simulink model "DATA_PERTURB_AND_OBSERVE_SOLAR_TRACKER"  (R2023b)
settings: Solver=ode23  StartTime=0.0  StopTime=12  RelTol=1e-7
undefined symbols (not defined in the file): Acid, Lead
libraries: spsMeanLib x5, spsSeriesRLCBranchLib x5, spsVoltageMeasurementLib x4, spsCurrentMeasurementLib x2, spsBatteryLib x1, spsDiodeLib x1, spsMosfetLib x1, simulink x1, spsPVArrayLib x1, spsPWMGeneratorDCDCLib x1, sps_lib x1
settings Model: Creator=User  LastModifiedBy=D E L L
settings DebuggingCC: AlgebraicLoopMsg=none

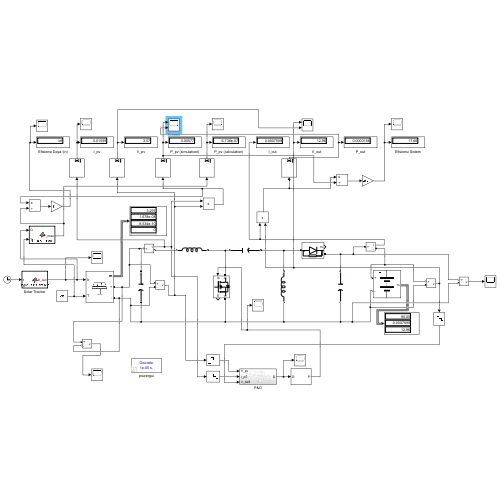
[thumbnail: Simulink's stored preview of the top-level diagram]
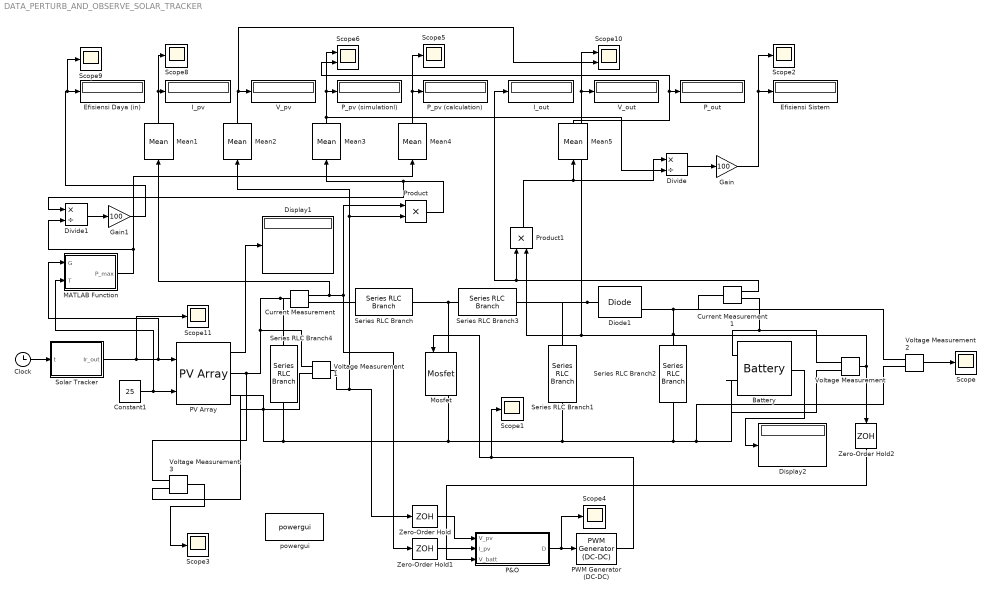
== system DATA_PERTURB_AND_OBSERVE_SOLAR_TRACKER ==
  Battery : spsBatteryLib/Battery  BatType=Lead-Acid  ShowTempParam=off  ThermalPreset=no  ShowAgeParam=off  NomV=12  NomQ=3.5  SOC=90  Batt_Tr=1  PresetModel=off  MaxQ=3.125  MinV=9  FullV=14.4  Dis_rate=0.6  R=0.04  Normal_OP=0.93083  expZone="[12.2171         0.01]"  current=[6.5 13 32.5]  Units=Time  Tci=20  NomT=20  T2=-30  MaxQ2=4.8  FullV2=7.1  Normal_OP2=5.655  expZone2="[6.58           1]"  Rca=0.6  ti=2000  Dp=0  Neq0=0  Tsim=1e6  Ta1=25  Qeol=5.4*0.9  Reol=0.013333*1.2  Char_age=[2.3478, 3]  Dis_age=[2.3478, 10]  N1=1500  N2=10500  N3=1000  N4=1400  Ta2=45  N5=950
  Clock : Clock
  Constant1 : Constant  Value=25
  Current Measurement : spsCurrentMeasurementLib/Current Measurement  PhasorSimulation=off  OutputType=Complex  PSBequivalent=0
  Current Measurement1 : spsCurrentMeasurementLib/Current Measurement  PhasorSimulation=off  OutputType=Complex  PSBequivalent=0
  Diode1 : spsDiodeLib/Diode  Ron=0.001  Lon=0  Vf=0.4  IC=0  UseSnubber=0  Rs=500  Cs=250e-9  Measurements=on
  Display1 : Display
  Display2 : Display
  Divide : Product  Inputs=*/
  Divide1 : Product  Inputs=*/
  Efisiensi Daya (in) : Display
  Efisiensi Sistem : Display
  Gain : Gain  Gain=100
  Gain1 : Gain  Gain=100
  I_out : Display
  I_pv : Display
  MATLAB Function : MATLAB Function  TreatAsAtomicUnit=on
  Mean{1..5} (5 alike) : spsMeanLib/Mean  Freq=60  Vinit=0  Ts=0
  Mosfet : spsMosfetLib/Mosfet  Ron=0.044  Lon=0  Rd=1.3  Vfd=0  IC=0  Rs=1e5  Cs=inf  Measurements=on
  P&O : Subsystem
  PV Array : spsPVArrayLib/PV Array  Npar=1  Nser=1  PlotType=array @ 1000 W/m2 & specified temperatures  S_vec="[ 1000  500  100 ]"  Temp_C_vec="[ 45 25  ]"  ModuleName=User-defined  PlotWhenSelected=off  Pm=10.08  Ncell=36  Voc=21.6  Isc=0.61  Vm=18  Im=0.56  beta_Voc_pc=-0.36099  alpha_Isc_pc=0.102  beta_Voc=-0.077974  alpha_Isc=0.0006222  IL=0.61115  I0=2.2544e-11  nI=0.97389  Rsh=828.4328  Rs=1.5603  RobustModel=off  RobustCellTemperature=313.3991  BAL=on  Tc=1e-6  Tfilter=1e-5
  PWM Generator (DC-DC) : spsPWMGeneratorDCDCLib/PWM Generator (DC-DC)  Fsw=31000  Ts=0
  P_out : Display
  P_pv (calculation) : Display
  P_pv (simulationl) : Display
  Product : Product
  Product1 : Product
  Scope{,1..5,8..9,11} (9 alike) : Scope
  Scope10 : Scope  NumInputPorts=2
  Scope6 : Scope  NumInputPorts=2
  Series RLC Branch : spsSeriesRLCBranchLib/Series RLC Branch  LConnTagsString=__new0  RConnTagsString=__new0  BranchType=L  Resistance=1  Inductance=1.5e-3  SetiL0=on  InitialCurrent=0.01  Capacitance=1e-6  Setx0=off  InitialVoltage=0  Measurements=None
  Series RLC Branch1 : spsSeriesRLCBranchLib/Series RLC Branch  LConnTagsString=__new0  RConnTagsString=__new0  BranchType=L  Resistance=1  Inductance=1.5e-3  SetiL0=on  InitialCurrent=0.01  Capacitance=1e-6  Setx0=off  InitialVoltage=0  Measurements=None
  Series RLC Branch2 : spsSeriesRLCBranchLib/Series RLC Branch  LConnTagsString=__new0  RConnTagsString=__new0  BranchType=C  Resistance=1  Inductance=1e-3  SetiL0=off  InitialCurrent=0  Capacitance=470e-6  Setx0=on  InitialVoltage=0.1  Measurements=None
  Series RLC Branch3 : spsSeriesRLCBranchLib/Series RLC Branch  LConnTagsString=__new0  RConnTagsString=__new0  BranchType=C  Resistance=1  Inductance=1e-3  SetiL0=off  InitialCurrent=0  Capacitance=22e-6  Setx0=off  InitialVoltage=0  Measurements=None
  Series RLC Branch4 : spsSeriesRLCBranchLib/Series RLC Branch  LConnTagsString=__new0  RConnTagsString=__new0  BranchType=C  Resistance=1  Inductance=1e-3  SetiL0=off  InitialCurrent=0  Capacitance=470e-6  Setx0=on  InitialVoltage=0.1  Measurements=None
  Solar Tracker : MATLAB Function  TreatAsAtomicUnit=on
  V_out : Display
  V_pv : Display
  Voltage Measurement{,1..3} (4 alike) : spsVoltageMeasurementLib/Voltage Measurement  PhasorSimulation=off  OutputType=Complex  PSBequivalent=0
  Zero-Order Hold : ZeroOrderHold  SampleTime=0.05
  Zero-Order Hold1 : ZeroOrderHold  SampleTime=0.05
  Zero-Order Hold2 : ZeroOrderHold  SampleTime=0.05
  powergui : sps_lib/powergui  Priority=1  SimulationMode=Discrete  SampleTime=1e-05  frequency=60  Iterations=50  frequencyindice=0  Pbase=100e6  ErrMax=1e-4  UnitsV=kV  UnitsW=MW  buscounter=0  FunctionMessages=off  echomessages=off  EnableUseOfTLC=off  CurrentSourceSwitches=off  DisableSnubberDevices=off  DisableRonSwitches=off  DisableVfSwitches=off  DisplayEquations=off  AutomaticDiscreteSolvers=off  SolverType=Tustin/Backward Euler (TBE)  Interpol=off  ExternalGateDelay=off  methode=off  Ts=100  x0status=blocks  SPID=on  SwTol=0  HookPort=off  NonlinearTolerance=1e-4  nMaxIteration=100  ContinueOnMaxIteration=off  RestoreLinks=warning  ResistiveCurrentMeasurement=off  Frange=[0:2:500]  Ylog=off  Xlog=on  ShowGrid=off  save=off  variable=ZData  structure=0  ZoomFFT=off  StartTime=0.0  cycles=1  DisplayStyle=1  fundamental=60  FreqAxis=off  MaxFrequency=1000  frequencyindicesteady=1  RmsSteady=1  display=off
  wires:
  Solar Tracker/1(Ir_out) -> Scope11/1, MATLAB Function/1(G), PV Array/1
  Constant1/1 -> MATLAB Function/2(T), PV Array/2
  PV Array/1 -> Display1/1
  Battery/1 -> Display2/1
  Voltage Measurement/1 -> Product1/2, Scope10/1, V_out/1, Zero-Order Hold2/1
  Voltage Measurement2/1 -> Scope/1
  Current Measurement/1 -> Zero-Order Hold1/1, Product/1, Mean1/1
  Voltage Measurement1/1 -> Zero-Order Hold/1, Mean2/1, Product/2
  PWM Generator (DC-DC)/1 -> Scope1/1, Mosfet/1
  Product/1 -> Mean3/1, Divide1/1
  Divide/1 -> Gain/1
  Current Measurement1/1 -> Product1/1, I_out/1
  Gain/1 -> Efisiensi Sistem/1, Scope2/1
  Product1/1 -> Divide/1, Mean5/1
  Mean4/1 -> Scope5/1, P_pv (calculation)/1
  Voltage Measurement3/1 -> Scope3/1
  MATLAB Function/1(P_max) -> Mean4/1, Divide1/2
  Divide1/1 -> Gain1/1
  Gain1/1 -> Scope9/1, Efisiensi Daya (in)/1
  Mean1/1 -> Scope8/1, I_pv/1
  Mean2/1 -> Scope10/2, V_pv/1
  Mean3/1 -> Scope6/1, P_pv (simulationl)/1, Divide/2
  Zero-Order Hold2/1 -> P&O/3(V_batt)
  Zero-Order Hold/1 -> P&O/1(V_pv)
  Zero-Order Hold1/1 -> P&O/2(I_pv)
  P&O/1(D) -> Scope4/1, PWM Generator (DC-DC)/1
  Clock/1 -> Solar Tracker/1(t)
  Mean5/1 -> Scope6/2, P_out/1
  connections:
  Diode1/LConn1 -- Series RLC Branch3/RConn1 -- Series RLC Branch1/LConn1
  Series RLC Branch2/LConn1 -- Current Measurement1/LConn1 -- Voltage Measurement2/LConn1 -- Diode1/RConn1
  Series RLC Branch1/RConn1 -- Series RLC Branch4/RConn1 -- Voltage Measurement3/LConn2 -- PV Array/RConn2 -- Voltage Measurement1/LConn2 -- Mosfet/RConn1 -- Voltage Measurement2/LConn2 -- Voltage Measurement/LConn2 -- Battery/LConn2 -- Series RLC Branch2/RConn1
  Current Measurement1/RConn1 -- Voltage Measurement/LConn1 -- Battery/LConn1
  Series RLC Branch3/LConn1 -- Series RLC Branch/RConn1 -- Mosfet/LConn1
  Current Measurement/RConn1 -- Series RLC Branch/LConn1
  PV Array/RConn1 -- Voltage Measurement3/LConn1 -- Voltage Measurement1/LConn1 -- Series RLC Branch4/LConn1 -- Current Measurement/LConn1

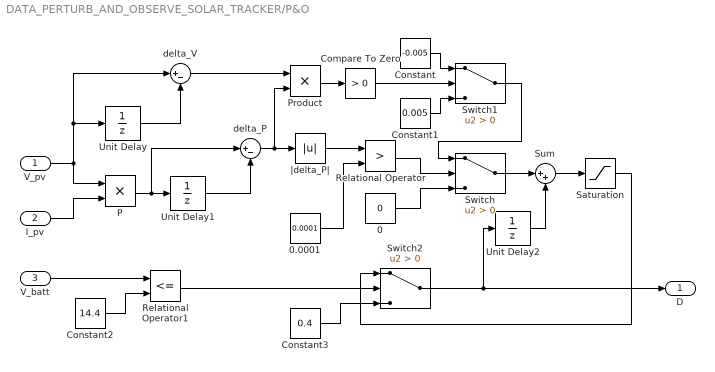
== system DATA_PERTURB_AND_OBSERVE_SOLAR_TRACKER/P&O ==
  V_pv : Inport
  I_pv : Inport  Port=2
  V_batt : Inport  Port=3
  0 : Constant  Value=0
  0.0001 : Constant  Value=0.0001
  Compare To Zero : simulink/Logic and Bit Operations/Compare To Zero  relop=>  OutDataTypeStr=boolean
  Constant : Constant  Value=-0.005
  Constant1 : Constant  Value=0.005
  Constant2 : Constant  Value=14.4
  Constant3 : Constant  Value=0.4
  P : Product
  Product : Product
  Relational Operator : RelationalOperator  Operator=>  OutDataTypeStr=boolean  RndMeth=Simplest  InputSameDT=off
  Relational Operator1 : RelationalOperator  Operator=<=  OutDataTypeStr=boolean  RndMeth=Simplest  InputSameDT=off
  Saturation : Saturate  UpperLimit=0.85  LowerLimit=0.15
  Sum : Sum  Inputs=|++
  Switch : Switch  Criteria=u2 > Threshold  SaturateOnIntegerOverflow=off  InputSameDT=off
  Switch1 : Switch  Criteria=u2 > Threshold  SaturateOnIntegerOverflow=off  InputSameDT=off
  Switch2 : Switch  Criteria=u2 > Threshold  SaturateOnIntegerOverflow=off  InputSameDT=off
  Unit Delay : UnitDelay  InitialCondition=21  SampleTime=-1  HasFrameUpgradeWarning=on
  Unit Delay1 : UnitDelay  SampleTime=-1  HasFrameUpgradeWarning=on
  Unit Delay2 : UnitDelay  InitialCondition=0.42  SampleTime=-1  HasFrameUpgradeWarning=on
  delta_P : Sum  Inputs=|+-
  delta_V : Sum  Inputs=|+-
  |delta_P| : Abs  SaturateOnIntegerOverflow=off
  D : Outport
  wires:
  Product/1 -> Compare To Zero/1
  Switch1/1 -> Switch/1
  Relational Operator1/1 -> Switch2/2
  Switch/1 -> Sum/1
  Switch2/1 -> D/1, Unit Delay2/1
  Constant2/1 -> Relational Operator1/2
  Saturation/1 -> Switch2/1
  Sum/1 -> Saturation/1
  delta_P/1 -> Product/2, |delta_P|/1
  Unit Delay2/1 -> Sum/2
  V_pv/1 -> P/1, delta_V/1, Unit Delay/1
  Constant1/1 -> Switch1/3
  delta_V/1 -> Product/1
  V_batt/1 -> Relational Operator1/1
  |delta_P|/1 -> Relational Operator/1
  0/1 -> Switch/3
  Unit Delay/1 -> delta_V/2
  I_pv/1 -> P/2
  Constant/1 -> Switch1/1
  Relational Operator/1 -> Switch/2
  Compare To Zero/1 -> Switch1/2
  P/1 -> delta_P/1, Unit Delay1/1
  0.0001/1 -> Relational Operator/2
  Constant3/1 -> Switch2/3
  Unit Delay1/1 -> delta_P/2

== matlab function DATA_PERTURB_AND_OBSERVE_SOLAR_TRACKER/MATLAB Function ==
  data: G input; P_max output; T input
function P_max = Pmax_Teori(G, T)
    % Parameter PV Array Piksel Liar / User-Defined
    P_stc = 10.08;   % Daya Maksimum (Watt)
    G_stc = 1000;    % Iradiasi standar (W/m^2)
    T_stc = 25;      % Suhu standar (Celcius)
    
    % Koefisien suhu untuk daya (dalam desimal)
    gamma = -0.0025899; 
    
    % Perhitungan Daya Maksimum Teoritis Dinamis
    P_max = P_stc * (G/G_stc) * (1 + gamma * (T - T_stc));
end

== matlab function DATA_PERTURB_AND_OBSERVE_SOLAR_TRACKER/Solar Tracker ==
  data: t input; Ir_out output
function Ir_out = single_axis_tracker(t)
    Ir_out = zeros(size(t));
    
    for i = 1:length(t)
        jam = 6 + t(i); 
        
        if jam > 6.001 && jam < 17.999 
            % --- 1. PARAMETER LOKASI ---
            phi = -7.77;           
            n = 81;                
            limit_rotasi = 60;     % Batas mekanis aktuator (derajat)
            
            % --- 2. GEOMETRI MATAHARI ---
            delta = 23.45 * sind(360 * (284 + n) / 365);
            omega = 15 * (jam - 12);
            
            sin_alpha = sind(phi)*sind(delta) + cosd(phi)*cosd(delta)*cosd(omega);
            alpha = asind(sin_alpha);
            
            if alpha > 0
                % --- 3. INTENSITAS CAHAYA (AM) ---
                I_o = 1367; 
                AM = 1 / (sind(alpha) + 0.00001); 
                DNI = I_o * 0.7 ^ (AM ^ 0.678); 
                
                % --- 4. LOGIKA SINGLE-AXIS TRACKER KONTINU ---
                % a. Hitung rotasi ideal yang dibutuhkan untuk mengejar matahari
                tan_rho = (cosd(delta) * sind(omega)) / sin_alpha;
                rho = atand(tan_rho);
                
                % b. Kemiringan panel (beta) adalah nilai absolut dari rho
                beta = abs(rho); 
                
                % c. SIMULASI MENTOK (Saturasi Aktuator)
                % Jika perhitungan ideal meminta panel miring lebih dari 60 derajat,
                % motor berhenti dan bertahan di kemiringan maksimumnya.
                if beta > limit_rotasi
                    beta = limit_rotasi;
                end
                
                % d. Penentuan Arah Hadap (Utara=180, Selatan=0 -> Timur=-90, Barat=90)
                if rho < 0
                    gamma = -90; % Menghadap Timur (Pagi)
                else
                    gamma = 90;  % Menghadap Barat (Sore)
                end
                
                % e. PERHITUNGAN COSINE LOSS (Satu rumus berlaku untuk semua kondisi)
                cos_theta = sind(phi)*sind(delta)*cosd(beta) ...
                          - cosd(phi)*sind(delta)*sind(beta)*cosd(gamma) ...
                          + cosd(phi)*cosd(delta)*cosd(beta)*cosd(omega) ...
                          + sind(phi)*cosd(delta)*sind(beta)*cosd(gamma)*cosd(omega) ...
                          + cosd(delta)*sind(beta)*sind(gamma)*sind(omega);
                          
                cos_theta = max(0, cos_theta);
                
                % --- 5. OUTPUT IRADIASI ---
                Ir_out(i) = DNI * cos_theta; 
            else
                Ir_out(i) = 0; 
            end
        else
            Ir_out(i) = 0; 
        end
    end
end
